simulink model "Main"  (R2025b)
settings: Solver=ode4  StartTime=0.0  StopTime=3600  FixedStep=0.1  RelTol=1e-3
values from neighbouring files (symbols this model uses):
  C1 = 17000    [Base.m]    (also in EKF_SOC_Estimator.m)
  C2 = 5200    [Base.m]
  OCV_tableData = ocv_data(:, 2)    [Base.m]
  Q_nominal = 50    [Base.m]
  R0 = 0.70 / 1000    (= 0.0007)    [Base.m]    (also in EKF_SOC_Estimator.m)
  R1 = 1.60 / 1000    (= 0.0016)    [Base.m]    (also in EKF_SOC_Estimator.m)
  R2 = 0.35 / 1000    (= 0.00035)    [Base.m]
  SOC_breakpoints = ocv_data(:, 1)    [Base.m]
undefined symbols (not defined in the file or in its folder): dspblkCoreblockFVToolHelper, gcbh
libraries: simulink x1
settings Model: Creator=Mohamed  LastModifiedBy=Mohamed

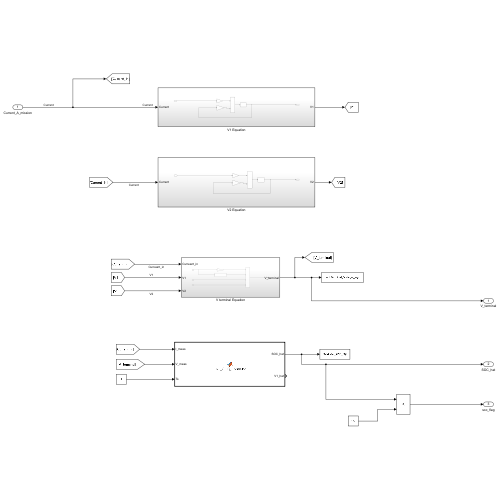
[thumbnail: Simulink's stored preview of the top-level diagram]
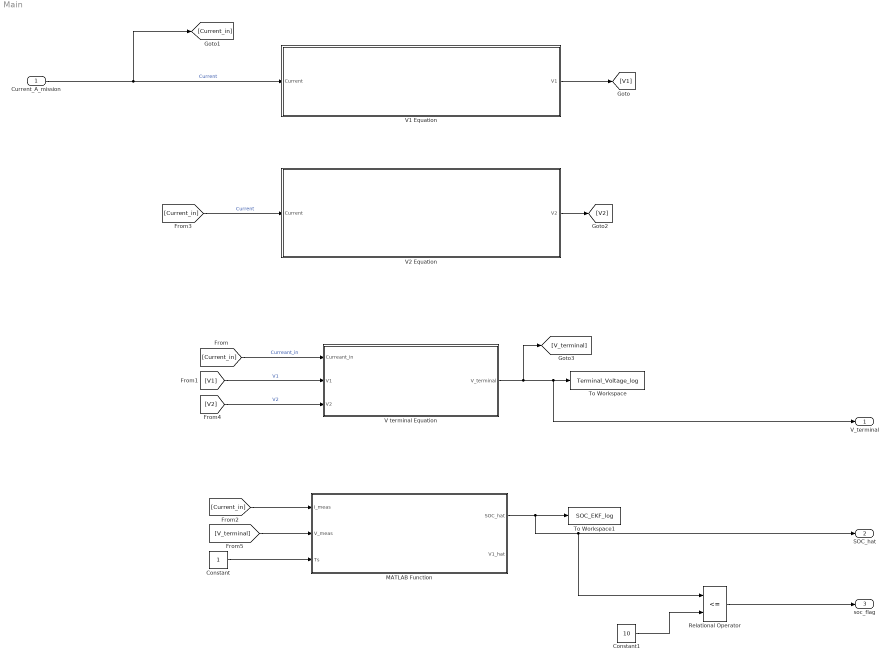
== system Main ==
  Current_A_mission : Inport
  Constant : Constant
  Constant1 : Constant  Value=10
  MATLAB Function : MATLAB Function  TreatAsAtomicUnit=on  SystemSampleTime=1
  Relational Operator : RelationalOperator  Operator=<=  OutDataTypeStr=boolean  RndMeth=Simplest  InputSameDT=off
  To Workspace : ToWorkspace  VariableName=Terminal_Voltage_log  SaveFormat=Structure With Time  SampleTime=-1
  To Workspace1 : ToWorkspace  VariableName=SOC_EKF_log  SaveFormat=Structure With Time  SampleTime=-1
  V terminal Equation : Subsystem
  V1 Equation : Subsystem
  V2 Equation : Subsystem
  V_terminal : Outport
  SOC_hat : Outport  Port=2
  soc_flag : Outport  Port=3
  wires:
  Current_A_mission/1 -> [Current_in], V1 Equation/1(Current)  "Current"
  V1 Equation/1(V1) -> [V1]
  [Current_in] -> V terminal Equation/1(Curreant_in)  "Curreant_in"
  [V1] -> V terminal Equation/2(V1)  "V1"
  V terminal Equation/1(V_terminal) -> [V_terminal], V_terminal/1, To Workspace/1
  [Current_in] -> V2 Equation/1(Current)  "Current"
  V2 Equation/1(V2) -> [V2]
  [V2] -> V terminal Equation/3(V2)  "V2"
  [Current_in] -> MATLAB Function/1(I_meas)
  [V_terminal] -> MATLAB Function/2(V_meas)
  Constant/1 -> MATLAB Function/3(Ts)
  MATLAB Function/1(SOC_hat) -> Relational Operator/1, SOC_hat/1, To Workspace1/1
  Constant1/1 -> Relational Operator/2
  Relational Operator/1 -> soc_flag/1

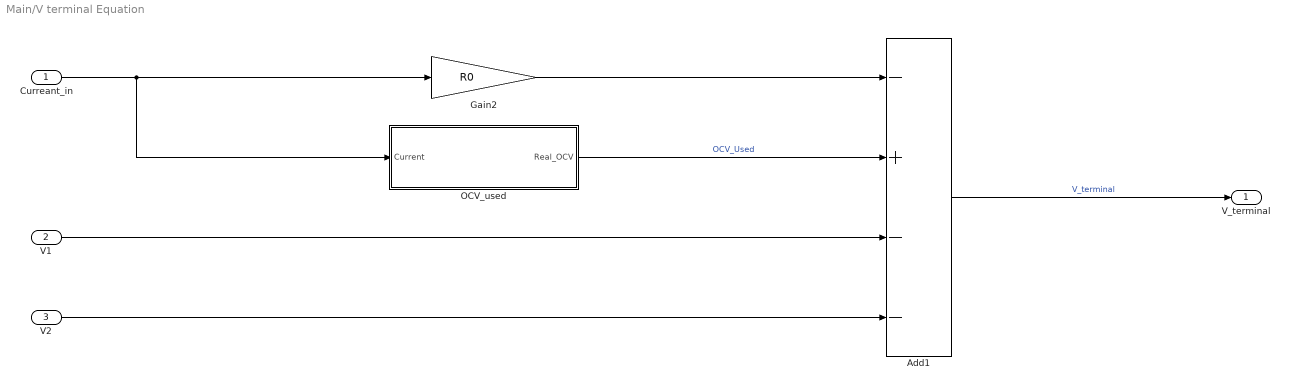
== system Main/V terminal Equation ==
  Curreant_in : Inport
  V1 : Inport  Port=2
  V2 : Inport  Port=3
  Add1 : Sum  Inputs=-+--
  Gain2 : Gain  Gain=R0
  OCV_used : Subsystem
  V_terminal : Outport
  wires:
  Curreant_in/1 -> Gain2/1, OCV_used/1(Current)
  Gain2/1 -> Add1/1
  Add1/1 -> V_terminal/1  "V_terminal"
  OCV_used/1(Real_OCV) -> Add1/2  "OCV_Used"
  V1/1 -> Add1/3
  V2/1 -> Add1/4

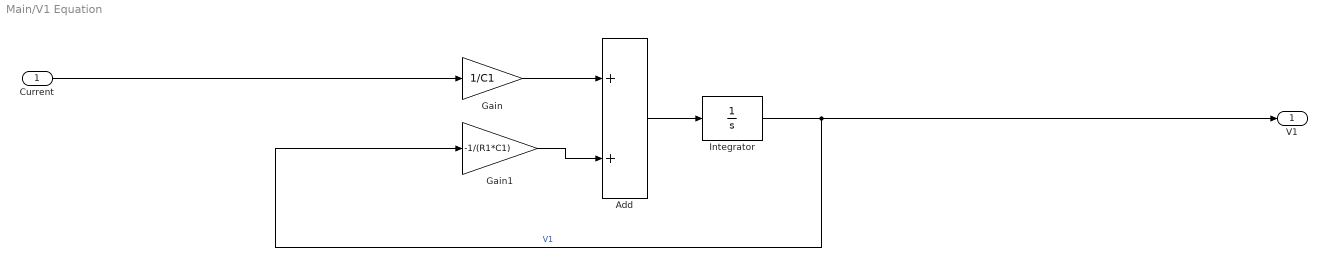
== system Main/V1 Equation ==
  Current : Inport
  Add : Sum
  Gain : Gain  Gain=1/C1
  Gain1 : Gain  Gain=-1/(R1*C1)
  Integrator : Integrator
  V1 : Outport
  wires:
  Integrator/1 -> V1/1, Gain1/1  "V1"
  Gain/1 -> Add/1
  Add/1 -> Integrator/1
  Current/1 -> Gain/1
  Gain1/1 -> Add/2

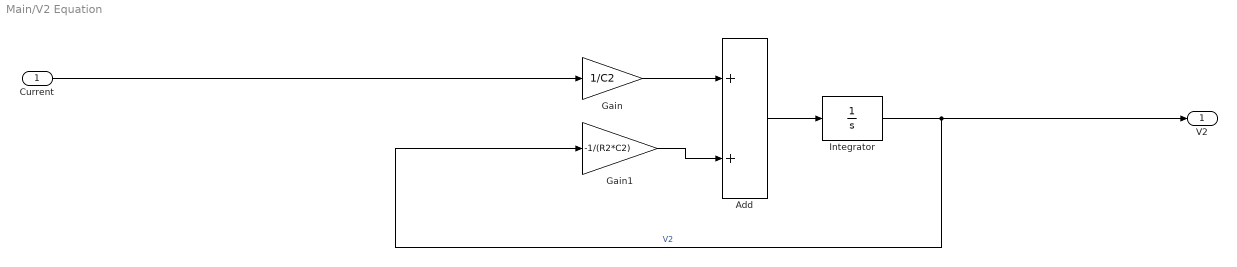
== system Main/V2 Equation ==
  Current : Inport
  Add : Sum
  Gain : Gain  Gain=1/C2
  Gain1 : Gain  Gain=-1/(R2*C2)
  Integrator : Integrator
  V2 : Outport
  wires:
  Gain1/1 -> Add/2
  Integrator/1 -> V2/1, Gain1/1  "V2"
  Add/1 -> Integrator/1
  Gain/1 -> Add/1
  Current/1 -> Gain/1

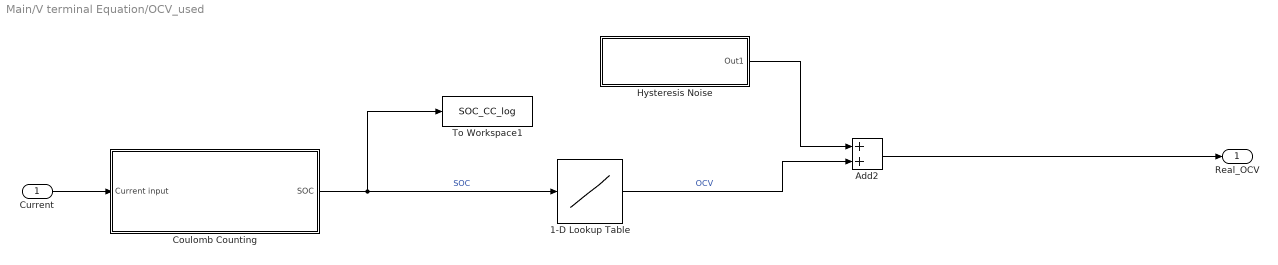
== system Main/V terminal Equation/OCV_used ==
  Current : Inport
  1-D Lookup Table : Lookup_n-D  NumberOfTableDimensions=1  BreakpointsForDimension1=SOC_breakpoints  Table=OCV_tableData  InternalRulePriority=Speed  RndMeth=Simplest
  Add2 : Sum
  Coulomb Counting : Subsystem
  Hysteresis Noise : Subsystem
  To Workspace1 : ToWorkspace  VariableName=SOC_CC_log  SaveFormat=Structure With Time  SampleTime=-1
  Real_OCV : Outport
  wires:
  Hysteresis Noise/1(Out1) -> Add2/1
  Current/1 -> Coulomb Counting/1(Current input)
  Coulomb Counting/1(SOC) -> To Workspace1/1, 1-D Lookup Table/1  "SOC"
  1-D Lookup Table/1 -> Add2/2  "OCV"
  Add2/1 -> Real_OCV/1

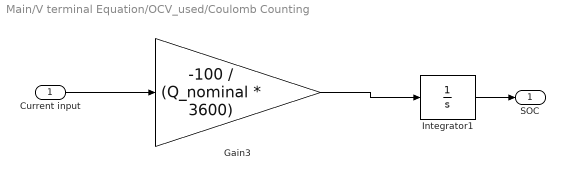
== system Main/V terminal Equation/OCV_used/Coulomb Counting ==
  Current input : Inport
  Gain3 : Gain  Gain=-100 / (Q_nominal * 3600)
  Integrator1 : Integrator  InitialCondition=80  LimitOutput=on  UpperSaturationLimit=90  LowerSaturationLimit=10
  SOC : Outport
  wires:
  Integrator1/1 -> SOC/1
  Gain3/1 -> Integrator1/1
  Current input/1 -> Gain3/1

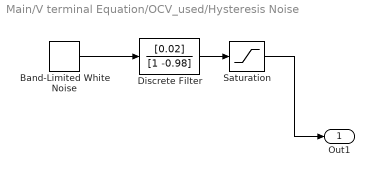
== system Main/V terminal Equation/OCV_used/Hysteresis Noise ==
  Band-Limited White Noise : simulink/Sources/Band-Limited White Noise  Cov=[1e-4]  Ts=1  seed=[23341]
  Discrete Filter : DiscreteFilter  LoadFcn=dspblkCoreblockFVToolHelper(gcbh,'load');  Numerator=[0.02]  Denominator=[1 -0.98]
      settings: CopyFcn=dspblkCoreblockFVToolHelper(gcbh,'copy');  DeleteFcn=dspblkCoreblockFVToolHelper(gcbh,'close');  ModelCloseFcn=dspblkCoreblockFVToolHelper(gcbh,'close');  PreSaveFcn=dspblkCoreblockFVToolHelper(gcbh,'presave');  PostSaveFcn=dspblkCoreblockFVToolHelper(gcbh,'postsave');  CloseFcn=dspblkCoreblockFVToolHelper(gcbh,'close');
  Saturation : Saturate  UpperLimit=0.005  LowerLimit=-0.005
  Out1 : Outport
  wires:
  Band-Limited White Noise/1 -> Discrete Filter/1
  Discrete Filter/1 -> Saturation/1
  Saturation/1 -> Out1/1

== matlab function Main/MATLAB Function ==
  data: I_meas input; SOC_hat output; V_meas input; Ts input; V1_hat output
function [SOC_hat, V1_hat] = EKF_SOC_Estimator(I_meas, V_meas, Ts)
%EKF_SOC_ESTIMATOR  Extended Kalman Filter SOC estimator for the Guardian
%   Battery ECM Project (1RC Thevenin model, LF50K 3.2V/50Ah LFP cell).
%
%   [SOC_hat, V1_hat] = EKF_SOC_Estimator(I_meas, V_meas, Ts)
%
%   Inputs:
%     I_meas  - measured cell current (A), discharge = POSITIVE
%     V_meas  - measured terminal voltage (V)
%     Ts      - sample time (s) -- must match the model's discrete step
%
%   Outputs:
%     SOC_hat - estimated state of charge (%)
%     V1_hat  - estimated RC-branch polarization voltage (V)
%
%   THIS FILE IS PROVIDED AS-IS. Do not modify the cell parameters,
%   OCV breakpoints, or filter structure -- only the noise tuning
%   (Qcov, Rcov) and initial covariance (P0) are meant to be adjusted
%   by students, and only if they can justify the change in their report.
%
%   Usage in Simulink: paste this exact function body into a MATLAB
%   Function block with two inputs (I_meas, V_meas) and two outputs
%   (SOC_hat, V1_hat). Pass Ts as a block mask parameter or hardcode it
%   to match your model's Fixed-Step discrete sample time.
%
%   Guardian Battery ECM Project - Part 2 Addendum
%   Reference cell parameters: see project datasheet, Appendix A.

%#codegen
persistent x P initialized
if isempty(initialized)
    x = [80; 0];            % initial state estimate [SOC(%); V1(V)]
                             % (80% matches the shared drive-cycle test's
                             % given initial condition -- do not change
                             % unless your report explains a cold-start
                             % scenario with an unknown initial SOC)
    P = diag([4, 0.01]);    % initial covariance
    initialized = true;
end

% ---- Fixed cell/model parameters (from project datasheet, Appendix A) ----
Q_nominal_Ah = 50;
R0 = 0.00070;      % ohm  (datasheet AC impedance, 1 kHz, mid-SOC, 25 C)
R1 = 0.00160;      % ohm  (scaled from literature HPPC fit, see Appendix A)
C1 = 17000;        % F
tau1 = R1 * C1;
a = exp(-Ts / tau1);

% ---- OCV-SOC breakpoints -- MUST match Guardian_Battery_OCV_SOC_Table.csv ----
soc_bp = [0 5 10 20 30 40 50 60 70 80 90 95 100];
ocv_bp = [2.50 2.95 3.05 3.15 3.20 3.22 3.24 3.26 3.28 3.30 3.33 3.45 3.65];

% ---- Process/measurement noise tuning ----
% Qcov reflects trust in the process model (SOC integration, V1 dynamics).
% Rcov reflects trust in the voltage measurement (~20 mV sensor noise assumed).
% Students may retune these two lines; document any change and why.
Qcov = diag([1e-3, 1e-6]);
Rcov = 4e-4;

% =====================================================================
% PREDICT
% =====================================================================
SOC_pred = x(1) - (Ts / (Q_nominal_Ah * 3600)) * I_meas * 100;
V1_pred  = a * x(2) + R1 * (1 - a) * I_meas;
x_pred = [SOC_pred; V1_pred];

F = [1, 0; 0, a];
P_pred = F * P * F' + Qcov;

% =====================================================================
% UPDATE
% =====================================================================
OCV_pred  = interp1(soc_bp, ocv_bp, x_pred(1), 'linear', 'extrap');

% Local OCV slope (finite-difference approximation of dOCV/dSOC at the
% predicted operating point) -- this is the nonlinear part of the EKF;
% a standard Kalman filter cannot handle this curved OCV(SOC) relationship.
d = 0.5;
dOCV_dSOC = interp1(soc_bp, ocv_bp, x_pred(1) + d, 'linear', 'extrap') ...
          - interp1(soc_bp, ocv_bp, x_pred(1) - d, 'linear', 'extrap');
dOCV_dSOC = dOCV_dSOC / (2 * d);

H = [dOCV_dSOC, -1];

V_pred = OCV_pred - I_meas * R0 - x_pred(2);
y_resid = V_meas - V_pred;

S = H * P_pred * H' + Rcov;
K = P_pred * H' / S;

x = x_pred + K * y_resid;
P = (eye(2) - K * H) * P_pred;

% Physical bound -- SOC cannot leave [0, 100]%
x(1) = min(max(x(1), 0), 100);

SOC_hat = x(1);
V1_hat  = x(2);

end
